simulink model "EMT_ML"  (R2024b)
settings: Solver=ode5  StartTime=0.0  StopTime=200  FixedStep=0.002  RelTol=1e-3
model workspace (MAT data in the model file):
  A = 7.3
  B = 2.71
  C0_shift = 200
  C1_shift = 200
  C2_shift = 200
  Cb = 70
  Cd = 0.6
  EMSInputBus : Simulink.Bus (value not decoded)
  Fb_max = 247500
  JA = 0.4
  JB = 0.4
  JZ = 0.4
  Jc1r2 = 0.01
  Jc3r4 = 0.01
  Jc4 = 0.01
  Je = 2.5
  Jh = 0.01
  Jq1 = 0.01
  Jq2 = 0.01
  Jr1 = 0.01
  Jr3s4 = 0.01
  Js123 = 0.01
  L = 4.472
  NE = [1600 1600 1600 1600 1600 1600 1600 1600 1600 1600 1600 1600 ... (840 elements, 30x28)]
  N_Te = 30
  N_ne = 28
  PE = [0 100.366530527 133.710336161 167.221698607 195.706356687 221.845219395 250.497434286 278.144308305 305.288511886 330.086920096 352.87464656 374.489475338 ... (840 elements, 30x28)]
  PN0 = 0
  Pb_epr = [-45 -45 -40 -30 0 30 40 45 45]
  Pb_max = [0 40 45 45 45]
  Pb_min = [-45 -45 -45 -40 0]
  Pe_ass = 230
  Pe_max = 1103
  Peg = [0 100 120 140 160 180 200 220 240 260 280 300 ... (53 elements, 1x53)]
  R_map = [0.09 0.089 0.09 0.091 0.092 0.093 0.094 0.095 0.096 0.097 0.098]
  SF_C0 = 1.5
  SF_C1 = 1.5
  SF_C2 = 1.5
  SF_Z1 = 1.5
  SF_Z2 = 1.5
  SF_ZD = 1.5
  SOC0 = 60
  SOC_epr = [30 31 50 59 60 61 70 79 80]
  SOC_map = [0 10 20 30 40 50 60 70 80 90 100]
  TA_max_map = [588.855 593.803361345 598.83559322 603.953846154 609.160344828 614.457391304 619.847368421 625.332743363 630.916071429 636.6 642.387272727 648.280733945 ... (115 elements, 1x115)]
  TA_min_map = [-588.855 -593.803361345 -598.83559322 -603.953846154 -609.160344828 -614.457391304 -619.847368421 -625.332743363 -630.916071429 -636.6 -642.387272727 -648.280733945 ... (115 elements, 1x115)]
  TAf = 0
  TB_max_map = [588.855 593.803361345 598.83559322 603.953846154 609.160344828 614.457391304 619.847368421 625.332743363 630.916071429 636.6 642.387272727 648.280733945 ... (115 elements, 1x115)]
  TB_min_map = [-588.855 -593.803361345 -598.83559322 -603.953846154 -609.160344828 -614.457391304 -619.847368421 -625.332743363 -630.916071429 -636.6 -642.387272727 -648.280733945 ... (115 elements, 1x115)]
  TBf = 0
  TE = [0 599 798 998 1168 1324 1495 1660 1822 1970 2106 2235 ... (840 elements, 30x28)]
  TS_A = 0.2
  TS_B = 0.2
  TS_C0 = 0.2
  TS_C1 = 0.2
  TS_C2 = 0.2
  TS_Z = 0.2
  TS_Z1 = 0.2
  TS_Z2 = 0.2
  TS_ZD = 0.2
  TZ_max_map = [537.13125 540.509433962 543.930379747 547.394904459 550.903846154 554.458064516 558.058441558 561.705882353 565.401315789 569.145695364 572.94 576.785234899 ... (131 elements, 1x131)]
  TZ_min_map = [-537.13125 -540.509433962 -543.930379747 -547.394904459 -550.903846154 -554.458064516 -558.058441558 -561.705882353 -565.401315789 -569.145695364 -572.94 -576.785234899 ... (131 elements, 1x131)]
  TZf = 0
  T_generator = [0 185 493.333333333 801.666666667 1110 1418.33333333 1726.66666667]
  T_motor = [0 185 493.333333333 801.666666667 1110 1418.33333333 1726.66666667]
  Te_map = [0 599 798 998 1168 1324 1495 1660 1822 1970 2106 2235 ... (30 elements, 1x30)]
  Te_max = 2754
  Te_max_map = [1168 1324 1495 1660 1822 1970 2106 2235 2355 2458 2543 2606 ... (28 elements, 1x28)]
  Te_start = 1600
  Tef = 100
  Teg = [0 596.8125 636.6 718.741935484 799.916230366 859.41 954.422788606 954.9 996.417391304 1078.98305085 1114.05 1169.26530612 ... (53 elements, 1x53)]
  Temax = 998
  Time = [0 0.1 0.2 0.3 0.4 0.5 0.6 0.7 0.8 0.9 1 1.1 ... (2001 elements, 1x2001)]
  Time_ele = [0 4 8 12 16 20 24 28 32 36 40 44 ... (401 elements, 1x401)]
  Time_fg = [0 2 4 6 8 10 12 14 16 18 20 22 ... (801 elements, 1x801)]
  Tmax_C0 = 2754
  Tmax_C1 = 3505.25455609
  Tmax_C2 = 3505.25455609
  Tmax_Z1 = 5584.80955498
  Tmax_Z2 = 16307.6439005
  Tmax_ZD = 3855.6
  Ts_e = 0.1
  Uoc_map = [814.5 917 933.25 945.75 958.25 969.25 978 985.25 993.25 1003.25 1050]
  V_Shift12 = 32
  V_Shift21 = 25
  V_Start = 10
  Voltage0 = 900
  Voltage_epr = [750 760 900 1000 1050]
  Y_engine = 0.955
  Yc = 0.98
  Yh = 0.96
  Yo = 0.92
  Yq = 0.94
  Z1_shift = 200
  Z2_shift = 200
  a11 = 1.54241568346
  a11_L = 1.54241568346
  a12 = -3.86074191629
  a12_L = 2.43173643789
  a21 = -1.04963112005
  a22 = 2.46948356808
  b11 = 0
  b11_L = 0
  b12 = 3.33
  b12_L = 7.8036
  b21 = 2.23571428571
  b22 = -2.13
  c11 = -0.648333656565
  c12 = 0
  c21 = -0.648333656565
  c22 = 0.680511182109
  controller_id = 1
  controller_name = 'Existing heuristic-grid EMS'
  cycle_grade = [0 0 0 0 0 0 0 0 0 0 0 0 ... (2001 elements, 1x2001)]
  cycle_road = [0.045 0.045 0.045 0.045 0.045 0.045 0.045 0.045 0.045 0.045 0.045 0.045 ... (2001 elements, 1x2001)]
  cycle_steering = [0 0 0 0 0 0 0 0 0 0 0 0 ... (2001 elements, 1x2001)]
  cycle_time = [0 0.1 0.2 0.3 0.4 0.5 0.6 0.7 0.8 0.9 1 1.1 ... (2001 elements, 1x2001)]
  d11 = -0.751666343435
  d12 = 0.3003003003
  d21 = -0.751666343435
  d22 = 0.319488817891
  e11 = -1.54241568346
  e12 = 0
  e21 = 1.04963112005
  e22 = -2.23571428571
  eff_generator = [0.8 0.8 0.79 0.79 0.76 0.74 0.72 0.8 0.85 0.88 0.85 0.8 ... (84 elements, 7x12)]
  eff_motor = [0.8 0.8 0.79 0.79 0.76 0.74 0.72 0.8 0.85 0.88 0.85 0.8 ... (84 elements, 7x12)]
  ele_map = [10 11.46 14.13 19.24 20.94 23.21 20.29 20.23 22.28 17.66 16.24 18.95 ... (401 elements, 1x401)]
  ems_runtime_config : object (value not decoded)
  f11 = -3.86074191629
  f12 = 3.33
  f21 = 2.46948356808
  f22 = -2.13
  fg = 0.045
  fg_map = [0.0125 0.0215 0.0332 0.0452 0.0525 0.0589 0.0584 0.0592 0.0621 0.0576 0.055 0.0572 ... (801 elements, 1x801)]
  fuel_gpkwh = [269.874826377 269.874826377 260.084605263 254.895150301 249.802821062 244.062054381 234.972466555 226.630558735 223.93243551 227.612775381 231.379615385 228.983738255 ... (840 elements, 30x28)]
  fuel_map = [269.874826377 269.874826377 260.084605263 254.895150301 249.802821062 244.062054381 234.972466555 226.630558735 223.93243551 227.612775381 231.379615385 228.983738255 ... (840 elements, 30x28)]
  fuel_map_N = [269.874826377 269.874826377 260.084605263 254.895150301 249.802821062 nan nan nan nan nan nan nan ... (840 elements, 30x28)]
  i = 28
  ic = 4.42
  iq = 1.4
  it = 4
  j = 30
  k1 = 2.13
  k2 = 2.13
  k3 = 2.33
  k4 = 1.92
  kh = 2.88
  kq = 2.17
  kt = 1.83
  mass = 45000
  miu_max = 0.8
  nA_map = [-6000 -5950 -5900 -5850 -5800 -5750 -5700 -5650 -5600 -5550 -5500 -5450 ... (115 elements, 1x115)]
  nA_max = 6000
  nA_min = -6000
  nB_map = [-6000 -5950 -5900 -5850 -5800 -5750 -5700 -5650 -5600 -5550 -5500 -5450 ... (115 elements, 1x115)]
  nB_max = 6000
  nB_min = -6000
  nB_start = 0
  nZ_map = [-8000 -7950 -7900 -7850 -7800 -7750 -7700 -7650 -7600 -7550 -7500 -7450 ... (131 elements, 1x131)]
  nZ_max = 8000
  nZ_min = -8000
  n_generator = [0 318.5 796.25 1274 1751.75 2229.5 2707.25 3185 3662.75 4140.5 4618.25 7007]
  n_motor = [0 318.5 796.25 1274 1751.75 2229.5 2707.25 3185 3662.75 4140.5 4618.25 7007]
  ne_idl = 3000
  ne_map = [1600 1700 1800 1900 2000 2100 2200 2300 2400 2500 2600 2700 ... (28 elements, 1x28)]
  ne_max = 4200
  ne_min = 1600
  ne_start = 200
  neg = [1600 1600 1800 1860 1910 2000 2001 2200 2300 2301 2400 2450 ... (53 elements, 1x53)]
  no_Shift12 = 1589.43589002
  no_Shift21 = 1241.74678908
  rz = 0.318
  startup_feedback_delay_s = 0.002
  startup_power_share = 0.5
  startup_speed_regularizer_rpm = 100
  v_cyc = [0 0 0 0 0 0 0 0 0 0 0 0 ... (2001 elements, 1x2001)]
  voltage_HighA = 1050
  voltage_HighB = 1050
  voltage_HighZ = 1050
  voltage_LowA = 750
  voltage_LowB = 750
  voltage_LowZ = 750
symbols that are objects in the model workspace (value not decoded): ems_runtime_config
undefined symbols (not defined in the file or in its folder): sigbuilder_block
libraries: fl_lib x82, nesl_utility x55, simulink x49, sdl_lib x10, slpidlib x3, simulink_need_slupdate x3, powerlib_extras x1
(part 5 of 7)

== system EMT_ML/Power Coupler /Z2/Z/Z2 ==
  Press : Inport
  Simulink-PS Converter : nesl_utility/Simulink-PS Converter  PhysicalDomain=network_engine_domain  SubClassName=ps_input  LeftPortType=input  RightPortType=output  PseudoPeriodic=off  Frequencies=[]  NoiseDistribution=none  NoiseParameters=[]  Unit=Pa  AffineConversion=off  FilteringAndDerivatives=filter  SimscapeFilterOrder=1  InputFilterTimeConstant=.001  UdotUserProvided=1
  Slip Sensor : Subsystem  mask(Slip Sensor){}
      mask help: The speed unit is r/min.
  Tire Radius2 : Gain  Gain=2500000
  Z2 : sdl_lib/Clutches/Disc Friction Clutch  geometry_model=2  r_eff=130 mm  d_o=189*2 mm  d_i=165.25*2 mm  nS=10  piston_area=0.0264 m^2  unidirectional=0  friction_model=1  mu_w_vector=[ 0 0.1 0.2 0.3 0.4 0.5 1 2 5 10 100 1000 ] rad/s  temperature_TLU=[280.0, 300.0, 320.0] K  mu_static=0.10  mu_static_vector=[0.4, 0.38, 0.36]  mu_coulomb=0.06  mu_coulomb_vector=[ 0.29 0.28 0.26 0.22 0.21 0.2 0.2 0.19 0.19 0.19 0.19 0.19 ]  mu_coulomb_temp_vector=[0.3, 0.28, 0.25]  mu_coulomb_matrix=[0.34, 0.32, 0.3; 0.3, 0.28, 0.25; 0.25, 0.2, 0.15]  mu_interp_method=1  mu_extrap_method=1  d_f=0.6  w_tol=0.001 rad/s  pressure_min=1830 Pa  mu_visc=0.0764 N*m/(rad/s)  initial_state_locked=0  thermal_mass=25 kJ/K  T_init=300 K
      settings: InternalSimscapePortConfiguration="{\"Bottom\":[],\"Left\":[{\"id\":\"P\",\"label\":\"P\",\"type\":\"input\"},{\"id\":\"B\",\"label\":\"B\",\"type\":\"foundation.mechanical.rotational.rotational\"}],\"Right\":[{\"id\":\"F\",\"label\":\"F\",\"type\":\"foundation.mechanical.rotational.rotational\"}],\"Top\":[]}"
  In : PMIOPort  Side=Left
  Out : PMIOPort  Port=2  Side=Right
  r/min : Outport
  wires:
  Slip Sensor/1(r/min) -> r/min/1
  Press/1 -> Tire Radius2/1
  Tire Radius2/1 -> Simulink-PS Converter/1
  connections:
  Slip Sensor/RConn1 -- Out/RConn1 -- Z2/RConn1
  Slip Sensor/LConn1 -- Z2/LConn2 -- In/RConn1
  Simulink-PS Converter/RConn1 -- Z2/LConn1

== system EMT_ML/Vehicle dynamics/vehicle dynamic/vehicle dynamic/Grade Resistance ==
  angle : Inport
  Ground Resistance : Fcn  Expr=0.5*mass*9.8*sin(u)
  Fg : Outport
  wires:
  Ground Resistance/1 -> Fg/1
  angle/1 -> Ground Resistance/1

== system EMT_ML/Vehicle dynamics/vehicle dynamic/vehicle dynamic/Ground Resistance ==
  fg : Inport
  angle : Inport  Port=2
  Ground Resistance : Fcn  Expr=0.5*u(1)*mass*9.8*cos(u(2))
  Mux : Mux  Inputs=2
  Ff : Outport
  wires:
  Ground Resistance/1 -> Ff/1
  Mux/1 -> Ground Resistance/1
  fg/1 -> Mux/1
  angle/1 -> Mux/2

== system EMT_ML/Vehicle dynamics/vehicle dynamic/vehicle dynamic/Mode Judge ==
  v : Inport
  Add : Sum  Inputs=+++
  Compare To Constant1 : simulink/Logic and Bit Operations/Compare To Constant  relop=<  const=-0.1  OutDataTypeStr=uint8
  Compare To Constant2 : simulink/Logic and Bit Operations/Compare To Constant  relop=>  const=0.1  OutDataTypeStr=uint8
  Compare To Constant3 : simulink/Logic and Bit Operations/Compare To Constant  relop=>=  const=-0.1  OutDataTypeStr=uint8
  Compare To Constant4 : simulink/Logic and Bit Operations/Compare To Constant  relop=<=  const=0.1  OutDataTypeStr=uint8
  Data Type Conversion : DataTypeConversion  SaturateOnIntegerOverflow=off  RndMeth=Floor
  Gain : Gain  Gain=3
  Gain1 : Gain  Gain=2
  Gain2 : Gain
  Logical Operator : Logic  AllPortsSameDT=off  OutDataTypeStr=boolean
  F : Outport
  wires:
  Gain1/1 -> Add/2
  Add/1 -> Data Type Conversion/1
  v/1 -> Compare To Constant4/1, Compare To Constant3/1, Compare To Constant2/1, Compare To Constant1/1
  Compare To Constant1/1 -> Gain2/1
  Compare To Constant3/1 -> Logical Operator/1
  Compare To Constant4/1 -> Logical Operator/2
  Compare To Constant2/1 -> Gain1/1
  Logical Operator/1 -> Gain/1
  Data Type Conversion/1 -> F/1
  Gain/1 -> Add/3
  Gain2/1 -> Add/1

== system EMT_ML/Vehicle dynamics/vehicle dynamic/vehicle dynamic/Speed Sensor ==
  Ideal Rotational Motion Sensor : fl_lib/Mechanical/Mechanical Sensors/Ideal Rotational Motion Sensor  reference=foundation.enum.MeasurementReference.difference  acceleration_port=false  velocity_port=true  position_port=true  wrap_angle=false  offset=0 rad
  PS-Simulink Converter : nesl_utility/PS-Simulink Converter  PhysicalDomain=network_engine_domain  SubClassName=ps_output  LeftPortType=input  RightPortType=output  PseudoPeriodic=off  Frequencies=[]  VectorFormat=1-D array  Unit=1  AffineConversion=off
  Reference : fl_lib/Mechanical/Rotational Elements/Mechanical Rotational Reference
  Tire Radius2 : Gain  Gain=30/pi
  shaft : PMIOPort  Side=Left
  r/min : Outport
  wires:
  Tire Radius2/1 -> r/min/1
  PS-Simulink Converter/1 -> Tire Radius2/1
  connections:
  shaft/RConn1 -- Ideal Rotational Motion Sensor/LConn1
  Reference/LConn1 -- Ideal Rotational Motion Sensor/RConn1
  PS-Simulink Converter/LConn1 -- Ideal Rotational Motion Sensor/RConn2

== system EMT_ML/Vehicle dynamics/vehicle dynamic/vehicle dynamic/Steering Resistance ==
  Abs : Abs  SaturateOnIntegerOverflow=off
  Compare To Constant : simulink/Logic and Bit Operations/Compare To Constant  relop=>=  const=10^3  OutDataTypeStr=uint8  ZeroCross=off
  Constant1 : Constant  Value=0
  Memory1 : Memory
  Memory3 : Memory
  Mux : Mux  Inputs=2
  Product2 : Product  RndMeth=Zero
  Sign1 : Signum
  Steering Resistance : Fcn  Expr=miu_max/(0.925+0.15*(u))*mass*9.8*L/4/B
  Switch : Switch  Threshold=1  SaturateOnIntegerOverflow=off  InputSameDT=off
  rou : Fcn  Expr=(u(1)+u(2))/(u(1)-u(2)+0.1^10)/2
  Fs : Outport
  wires:
  Steering Resistance/1 -> Product2/1
  Memory3/1 -> Mux/1
  Memory1/1 -> Mux/2
  Mux/1 -> rou/1
  rou/1 -> Abs/1, Compare To Constant/1, Sign1/1
  Abs/1 -> Steering Resistance/1  "rou"
  Compare To Constant/1 -> Switch/2
  Constant1/1 -> Switch/1
  Switch/1 -> Product2/2
  Sign1/1 -> Switch/3
  Product2/1 -> Fs/1
  [v_Left] -> Memory3/1
  [v_Right] -> Memory1/1

== system EMT_ML/Vehicle dynamics/vehicle dynamic/vehicle dynamic/Torque Actuator ==
  torque : Inport
  Ideal Torque Source : fl_lib/Mechanical/Mechanical Sources/Ideal Torque Source
  Mechanical Rotational Reference : fl_lib/Mechanical/Rotational Elements/Mechanical Rotational Reference
  Simulink-PS Converter : nesl_utility/Simulink-PS Converter  PhysicalDomain=network_engine_domain  SubClassName=ps_input  LeftPortType=input  RightPortType=output  PseudoPeriodic=off  Frequencies=[]  NoiseDistribution=none  NoiseParameters=[]  Unit=1  AffineConversion=off  FilteringAndDerivatives=filter  SimscapeFilterOrder=2  InputFilterTimeConstant=.001  UdotUserProvided=1
  shaft : PMIOPort  Side=Right
  wires:
  torque/1 -> Simulink-PS Converter/1
  connections:
  Simulink-PS Converter/RConn1 -- Ideal Torque Source/RConn1
  Mechanical Rotational Reference/LConn1 -- Ideal Torque Source/RConn2
  shaft/RConn1 -- Ideal Torque Source/LConn1

== system EMT_ML/Vehicle dynamics/vehicle dynamic/vehicle dynamic/Torque Sensor ==
  Ideal Torque Sensor : fl_lib/Mechanical/Mechanical Sensors/Ideal Torque Sensor
  PS-Simulink Converter : nesl_utility/PS-Simulink Converter  PhysicalDomain=network_engine_domain  SubClassName=ps_output  LeftPortType=input  RightPortType=output  PseudoPeriodic=off  Frequencies=[]  VectorFormat=1-D array  Unit=1  AffineConversion=off
  In : PMIOPort  Side=Left
  Out : PMIOPort  Port=2  Side=Right
  Nm : Outport
  wires:
  PS-Simulink Converter/1 -> Nm/1
  connections:
  PS-Simulink Converter/LConn1 -- Ideal Torque Sensor/RConn2
  In/RConn1 -- Ideal Torque Sensor/LConn1
  Ideal Torque Sensor/RConn1 -- Out/RConn1

== system EMT_ML/Vehicle dynamics/vehicle dynamic/vehicle dynamic/Wind Resistance ==
  Air Resistance : Fcn  Expr=0.5*Cd*A*u*u/21.15
  Memory3 : Memory
  Fw : Outport
  wires:
  [v_act] -> Memory3/1
  Memory3/1 -> Air Resistance/1
  Air Resistance/1 -> Fw/1

== system EMT_ML/Vehicle dynamics/vehicle dynamic/vehicle dynamic1/Grade Resistance ==
  angle : Inport
  Ground Resistance : Fcn  Expr=0.5*mass*9.8*sin(u)
  Fg : Outport
  wires:
  angle/1 -> Ground Resistance/1
  Ground Resistance/1 -> Fg/1

== system EMT_ML/Vehicle dynamics/vehicle dynamic/vehicle dynamic1/Ground Resistance ==
  fg : Inport
  angle : Inport  Port=2
  Ground Resistance : Fcn  Expr=0.5*u(1)*mass*9.8*cos(u(2))
  Mux : Mux  Inputs=2
  Ff : Outport
  wires:
  angle/1 -> Mux/2
  fg/1 -> Mux/1
  Mux/1 -> Ground Resistance/1
  Ground Resistance/1 -> Ff/1

== system EMT_ML/Vehicle dynamics/vehicle dynamic/vehicle dynamic1/Mode Judge ==
  v : Inport
  Add : Sum  Inputs=+++
  Compare To Constant1 : simulink/Logic and Bit Operations/Compare To Constant  relop=<  const=-0.1  OutDataTypeStr=uint8
  Compare To Constant2 : simulink/Logic and Bit Operations/Compare To Constant  relop=>  const=0.1  OutDataTypeStr=uint8
  Compare To Constant3 : simulink/Logic and Bit Operations/Compare To Constant  relop=>=  const=-0.1  OutDataTypeStr=uint8
  Compare To Constant4 : simulink/Logic and Bit Operations/Compare To Constant  relop=<=  const=0.1  OutDataTypeStr=uint8
  Data Type Conversion : DataTypeConversion  SaturateOnIntegerOverflow=off  RndMeth=Floor
  Gain : Gain  Gain=3
  Gain1 : Gain  Gain=2
  Gain2 : Gain
  Logical Operator : Logic  AllPortsSameDT=off  OutDataTypeStr=boolean
  F : Outport
  wires:
  Gain2/1 -> Add/1
  Gain/1 -> Add/3
  Data Type Conversion/1 -> F/1
  Logical Operator/1 -> Gain/1
  Compare To Constant2/1 -> Gain1/1
  Compare To Constant4/1 -> Logical Operator/2
  Compare To Constant3/1 -> Logical Operator/1
  Compare To Constant1/1 -> Gain2/1
  v/1 -> Compare To Constant1/1, Compare To Constant2/1, Compare To Constant3/1, Compare To Constant4/1
  Add/1 -> Data Type Conversion/1
  Gain1/1 -> Add/2

== system EMT_ML/Vehicle dynamics/vehicle dynamic/vehicle dynamic1/Speed Sensor ==
  Ideal Rotational Motion Sensor : fl_lib/Mechanical/Mechanical Sensors/Ideal Rotational Motion Sensor  reference=foundation.enum.MeasurementReference.difference  acceleration_port=false  velocity_port=true  position_port=true  wrap_angle=false  offset=0 rad
  PS-Simulink Converter : nesl_utility/PS-Simulink Converter  PhysicalDomain=network_engine_domain  SubClassName=ps_output  LeftPortType=input  RightPortType=output  PseudoPeriodic=off  Frequencies=[]  VectorFormat=1-D array  Unit=1  AffineConversion=off
  Reference : fl_lib/Mechanical/Rotational Elements/Mechanical Rotational Reference
  Tire Radius2 : Gain  Gain=30/pi
  shaft : PMIOPort  Side=Left
  r/min : Outport
  wires:
  PS-Simulink Converter/1 -> Tire Radius2/1
  Tire Radius2/1 -> r/min/1
  connections:
  PS-Simulink Converter/LConn1 -- Ideal Rotational Motion Sensor/RConn2
  Reference/LConn1 -- Ideal Rotational Motion Sensor/RConn1
  shaft/RConn1 -- Ideal Rotational Motion Sensor/LConn1

== system EMT_ML/Vehicle dynamics/vehicle dynamic/vehicle dynamic1/Steering Resistance ==
  Abs : Abs  SaturateOnIntegerOverflow=off
  Compare To Constant : simulink/Logic and Bit Operations/Compare To Constant  relop=>=  const=10^3  OutDataTypeStr=uint8  ZeroCross=off
  Constant1 : Constant  Value=0
  Memory1 : Memory
  Memory3 : Memory
  Mux : Mux  Inputs=2
  Product2 : Product  RndMeth=Zero
  Sign1 : Signum
  Steering Resistance : Fcn  Expr=miu_max/(0.925+0.15*(u))*mass*9.8*L/4/B
  Switch : Switch  Threshold=1  SaturateOnIntegerOverflow=off  InputSameDT=off
  rou : Fcn  Expr=(u(1)+u(2))/(u(2)-u(1)+0.1^10)/2
  Fs : Outport
  wires:
  [v_Right] -> Memory1/1
  [v_Left] -> Memory3/1
  Product2/1 -> Fs/1
  Sign1/1 -> Switch/3
  Switch/1 -> Product2/2
  Constant1/1 -> Switch/1
  Compare To Constant/1 -> Switch/2
  Abs/1 -> Steering Resistance/1  "rou"
  rou/1 -> Sign1/1, Compare To Constant/1, Abs/1
  Mux/1 -> rou/1
  Memory1/1 -> Mux/2
  Memory3/1 -> Mux/1
  Steering Resistance/1 -> Product2/1

== system EMT_ML/Vehicle dynamics/vehicle dynamic/vehicle dynamic1/Torque Actuator ==
  torque : Inport
  Ideal Torque Source : fl_lib/Mechanical/Mechanical Sources/Ideal Torque Source
  Mechanical Rotational Reference : fl_lib/Mechanical/Rotational Elements/Mechanical Rotational Reference
  Simulink-PS Converter : nesl_utility/Simulink-PS Converter  PhysicalDomain=network_engine_domain  SubClassName=ps_input  LeftPortType=input  RightPortType=output  PseudoPeriodic=off  Frequencies=[]  NoiseDistribution=none  NoiseParameters=[]  Unit=1  AffineConversion=off  FilteringAndDerivatives=filter  SimscapeFilterOrder=2  InputFilterTimeConstant=.001  UdotUserProvided=1
  shaft : PMIOPort  Side=Right
  wires:
  torque/1 -> Simulink-PS Converter/1
  connections:
  shaft/RConn1 -- Ideal Torque Source/LConn1
  Mechanical Rotational Reference/LConn1 -- Ideal Torque Source/RConn2
  Simulink-PS Converter/RConn1 -- Ideal Torque Source/RConn1

== system EMT_ML/Vehicle dynamics/vehicle dynamic/vehicle dynamic1/Torque Sensor ==
  Ideal Torque Sensor : fl_lib/Mechanical/Mechanical Sensors/Ideal Torque Sensor
  PS-Simulink Converter : nesl_utility/PS-Simulink Converter  PhysicalDomain=network_engine_domain  SubClassName=ps_output  LeftPortType=input  RightPortType=output  PseudoPeriodic=off  Frequencies=[]  VectorFormat=1-D array  Unit=1  AffineConversion=off
  In : PMIOPort  Side=Left
  Out : PMIOPort  Port=2  Side=Right
  Nm : Outport
  wires:
  PS-Simulink Converter/1 -> Nm/1
  connections:
  Ideal Torque Sensor/RConn1 -- Out/RConn1
  In/RConn1 -- Ideal Torque Sensor/LConn1
  PS-Simulink Converter/LConn1 -- Ideal Torque Sensor/RConn2

== system EMT_ML/Vehicle dynamics/vehicle dynamic/vehicle dynamic1/Wind Resistance ==
  Air Resistance : Fcn  Expr=0.5*Cd*A*u*u/21.15
  Memory3 : Memory
  Fw : Outport
  wires:
  [v_act] -> Memory3/1
  Memory3/1 -> Air Resistance/1
  Air Resistance/1 -> Fw/1

== system EMT_ML/engine/Engine/Subsystem1/Torque Actuator ==
  torque : Inport
  Ideal Torque Source : fl_lib/Mechanical/Mechanical Sources/Ideal Torque Source
  Mechanical Rotational Reference : fl_lib/Mechanical/Rotational Elements/Mechanical Rotational Reference
  Simulink-PS Converter : nesl_utility/Simulink-PS Converter  PhysicalDomain=network_engine_domain  SubClassName=ps_input  LeftPortType=input  RightPortType=output  PseudoPeriodic=off  Frequencies=[]  NoiseDistribution=none  NoiseParameters=[]  Unit=N*m  AffineConversion=off  FilteringAndDerivatives=zero  SimscapeFilterOrder=1  InputFilterTimeConstant=.001  UdotUserProvided=0
  shaft : PMIOPort  Side=Right
  wires:
  torque/1 -> Simulink-PS Converter/1
  connections:
  Simulink-PS Converter/RConn1 -- Ideal Torque Source/RConn1
  Mechanical Rotational Reference/LConn1 -- Ideal Torque Source/RConn2
  shaft/RConn1 -- Ideal Torque Source/LConn1

== system EMT_ML/motorA/Motor/Mechanical Body/Max & Min Torque Control ==
  speed : Inport
  Tm_com : Inport  Port=2
  Lookup Table : Lookup  InputValues=nm_map  Table=Tm_max_map  SaturateOnIntegerOverflow=off
  Lookup Table1 : Lookup  InputValues=nm_map  Table=Tm_min_map  SaturateOnIntegerOverflow=off
  Saturation Dynamic : simulink/Discontinuities/Saturation Dynamic  OutMin=[]  OutMax=[]  OutDataTypeStr=Inherit: Same as second input  OutDataType=sfix(16)  OutScaling=2^-10  DoSatur=off
  Saturation1 : Saturate  UpperLimit=max(nm_map)  LowerLimit=min(nm_map)
  Saturation2 : Saturate  UpperLimit=max(nm_map)  LowerLimit=min(nm_map)
  Transfer Fcn : TransferFcn  Denominator=[T 1]
  torque : Outport
  wires:
  speed/1 -> Saturation2/1, Saturation1/1
  Lookup Table/1 -> Saturation Dynamic/1
  Lookup Table1/1 -> Saturation Dynamic/3
  Saturation1/1 -> Lookup Table/1
  Saturation2/1 -> Lookup Table1/1
  Tm_com/1 -> Saturation Dynamic/2
  Saturation Dynamic/1 -> Transfer Fcn/1
  Transfer Fcn/1 -> torque/1

== system EMT_ML/motorA/Motor/Mechanical Body/Resistance ==
  speed : Inport
  Constant2 : Constant  Value=-Tmf
  Product2 : Product  RndMeth=Zero
  Sign2 : Signum
  Torque Actuator : Subsystem  mask(Torque Actuator){}
      mask help: The torque unit is Nm.
  Tmf : PMIOPort  Side=Right
  wires:
  speed/1 -> Sign2/1
  Product2/1 -> Torque Actuator/1(torque)
  Sign2/1 -> Product2/1
  Constant2/1 -> Product2/2
  connections:
  Tmf/RConn1 -- Torque Actuator/RConn1

== system EMT_ML/motorA/Motor/Mechanical Body/Speed Sensor ==
  Ideal Rotational Motion Sensor : fl_lib/Mechanical/Mechanical Sensors/Ideal Rotational Motion Sensor  reference=foundation.enum.MeasurementReference.difference  acceleration_port=false  velocity_port=true  position_port=true  wrap_angle=false  offset=0 rad
  PS-Simulink Converter : nesl_utility/PS-Simulink Converter  PhysicalDomain=network_engine_domain  SubClassName=ps_output  LeftPortType=input  RightPortType=output  PseudoPeriodic=off  Frequencies=[]  VectorFormat=1-D array  Unit=rad/s  AffineConversion=off
  Reference : fl_lib/Mechanical/Rotational Elements/Mechanical Rotational Reference
  Tire Radius2 : Gain  Gain=30/pi
  shaft : PMIOPort  Side=Left
  r/min : Outport
  wires:
  Tire Radius2/1 -> r/min/1
  PS-Simulink Converter/1 -> Tire Radius2/1
  connections:
  shaft/RConn1 -- Ideal Rotational Motion Sensor/LConn1
  Reference/LConn1 -- Ideal Rotational Motion Sensor/RConn1
  PS-Simulink Converter/LConn1 -- Ideal Rotational Motion Sensor/RConn2

== system EMT_ML/motorA/Motor/Mechanical Body/Torque Actuator ==
  torque : Inport
  Ideal Torque Source : fl_lib/Mechanical/Mechanical Sources/Ideal Torque Source
  Mechanical Rotational Reference : fl_lib/Mechanical/Rotational Elements/Mechanical Rotational Reference
  Simulink-PS Converter : nesl_utility/Simulink-PS Converter  PhysicalDomain=network_engine_domain  SubClassName=ps_input  LeftPortType=input  RightPortType=output  PseudoPeriodic=off  Frequencies=[]  NoiseDistribution=none  NoiseParameters=[]  Unit=N*m  AffineConversion=off  FilteringAndDerivatives=filter  SimscapeFilterOrder=1  InputFilterTimeConstant=.001  UdotUserProvided=1
  shaft : PMIOPort  Side=Right
  wires:
  torque/1 -> Simulink-PS Converter/1
  connections:
  shaft/RConn1 -- Ideal Torque Source/LConn1
  Mechanical Rotational Reference/LConn1 -- Ideal Torque Source/RConn2
  Simulink-PS Converter/RConn1 -- Ideal Torque Source/RConn1

== system EMT_ML/motorB/Motor/Mechanical Body/Max & Min Speed Control ==
  speed : Inport
  Tm_com : Inport  Port=2
  Lookup Table : Lookup  InputValues=nm_map  Table=Tm_max_map  SaturateOnIntegerOverflow=off
  Lookup Table1 : Lookup  InputValues=nm_map  Table=Tm_min_map  SaturateOnIntegerOverflow=off
  Saturation Dynamic : simulink/Discontinuities/Saturation Dynamic  OutMin=[]  OutMax=[]  OutDataTypeStr=Inherit: Same as second input  OutDataType=sfix(16)  OutScaling=2^-10  DoSatur=off
  Saturation1 : Saturate  UpperLimit=max(nm_map)  LowerLimit=min(nm_map)
  Saturation2 : Saturate  UpperLimit=max(nm_map)  LowerLimit=min(nm_map)
  Transfer Fcn : TransferFcn  Denominator=[T 1]
  torque : Outport
  wires:
  Transfer Fcn/1 -> torque/1
  speed/1 -> Saturation2/1, Saturation1/1
  Lookup Table/1 -> Saturation Dynamic/1
  Lookup Table1/1 -> Saturation Dynamic/3
  Saturation1/1 -> Lookup Table/1
  Saturation2/1 -> Lookup Table1/1
  Tm_com/1 -> Saturation Dynamic/2
  Saturation Dynamic/1 -> Transfer Fcn/1

== system EMT_ML/motorB/Motor/Mechanical Body/Resistance ==
  speed : Inport
  Constant2 : Constant  Value=-Tmf
  Product2 : Product  RndMeth=Zero
  Sign2 : Signum
  Torque Actuator : Subsystem  mask(Torque Actuator){}
      mask help: The torque unit is Nm.
  Tmf : PMIOPort  Side=Right
  wires:
  speed/1 -> Sign2/1
  Product2/1 -> Torque Actuator/1(torque)
  Sign2/1 -> Product2/1
  Constant2/1 -> Product2/2
  connections:
  Tmf/RConn1 -- Torque Actuator/RConn1

== system EMT_ML/motorB/Motor/Mechanical Body/Speed Sensor ==
  Ideal Rotational Motion Sensor : fl_lib/Mechanical/Mechanical Sensors/Ideal Rotational Motion Sensor  reference=foundation.enum.MeasurementReference.difference  acceleration_port=false  velocity_port=true  position_port=true  wrap_angle=false  offset=0 rad
  PS-Simulink Converter : nesl_utility/PS-Simulink Converter  PhysicalDomain=network_engine_domain  SubClassName=ps_output  LeftPortType=input  RightPortType=output  PseudoPeriodic=off  Frequencies=[]  VectorFormat=1-D array  Unit=rad/s  AffineConversion=off
  Reference : fl_lib/Mechanical/Rotational Elements/Mechanical Rotational Reference
  Tire Radius2 : Gain  Gain=30/pi
  shaft : PMIOPort  Side=Left
  r/min : Outport
  wires:
  Tire Radius2/1 -> r/min/1
  PS-Simulink Converter/1 -> Tire Radius2/1
  connections:
  shaft/RConn1 -- Ideal Rotational Motion Sensor/LConn1
  Reference/LConn1 -- Ideal Rotational Motion Sensor/RConn1
  PS-Simulink Converter/LConn1 -- Ideal Rotational Motion Sensor/RConn2

== system EMT_ML/motorB/Motor/Mechanical Body/Torque Actuator ==
  torque : Inport
  Ideal Torque Source : fl_lib/Mechanical/Mechanical Sources/Ideal Torque Source
  Mechanical Rotational Reference : fl_lib/Mechanical/Rotational Elements/Mechanical Rotational Reference
  Simulink-PS Converter : nesl_utility/Simulink-PS Converter  PhysicalDomain=network_engine_domain  SubClassName=ps_input  LeftPortType=input  RightPortType=output  PseudoPeriodic=off  Frequencies=[]  NoiseDistribution=none  NoiseParameters=[]  Unit=N*m  AffineConversion=off  FilteringAndDerivatives=filter  SimscapeFilterOrder=1  InputFilterTimeConstant=.001  UdotUserProvided=1
  shaft : PMIOPort  Side=Right
  wires:
  torque/1 -> Simulink-PS Converter/1
  connections:
  shaft/RConn1 -- Ideal Torque Source/LConn1
  Mechanical Rotational Reference/LConn1 -- Ideal Torque Source/RConn2
  Simulink-PS Converter/RConn1 -- Ideal Torque Source/RConn1

== system EMT_ML/Control Unit/Control/EVT1_H Stage/clutches condition/Subsystem ==
  Constant1 : Constant
  C0 : Outport
  wires:
  Constant1/1 -> C0/1

== system EMT_ML/Control Unit/Control/EVT1_H Stage/clutches condition/Subsystem1 ==
  Constant1 : Constant
  Z2 : Outport
  wires:
  Constant1/1 -> Z2/1

== system EMT_ML/Control Unit/Control/EVT1_H Stage/clutches condition/Subsystem2 ==
  Compare To Constant1 : simulink/Logic and Bit Operations/Compare To Constant  relop=<  const=C1_shift  OutDataTypeStr=uint8
  Data Type Conversion : DataTypeConversion  SaturateOnIntegerOverflow=off  RndMeth=Floor
  Fcn : Fcn  Expr=V_Shift12+5*(u-1)
  Logical Operator1 : Logic  AllPortsSameDT=off  OutDataTypeStr=boolean
  Memory1 : Memory
  Memory2 : Memory
  Memory5 : Memory
  Relational Operator : RelationalOperator  OutDataTypeStr=boolean  InputSameDT=off
  C1 : Outport
  wires:
  Logical Operator1/1 -> Data Type Conversion/1
  Compare To Constant1/1 -> Logical Operator1/2
  Relational Operator/1 -> Logical Operator1/1
  Fcn/1 -> Relational Operator/2
  Memory1/1 -> Fcn/1
  [Acc_pedal] -> Memory1/1
  Memory2/1 -> Relational Operator/1
  Memory5/1 -> Compare To Constant1/1
  [C1_rela] -> Memory5/1
  Data Type Conversion/1 -> C1/1
  [v_act] -> Memory2/1

== system EMT_ML/Control Unit/Control/EVT1_H Stage/clutches condition/Subsystem4 ==
  Constant1 : Constant  Value=0
  Z1 : Outport
  wires:
  Constant1/1 -> Z1/1

== system EMT_ML/Control Unit/Control/EVT1_H Stage/engine torque/Subsystem1 ==
  Te_ref : Inport
  ne_act : Inport  Port=2
  Constant : Constant  Value=ne_idl
  Constant1 : Constant  Value=0
  Lookup Table : Lookup  InputValues=ne_map  Table=Te_max_map  SaturateOnIntegerOverflow=off
  Memory1 : Memory
  Memory5 : Memory
  PID Controller2 : slpidlib/PID Controller  Controller=PID  Form=Parallel  TimeDomain=Continuous-time  UseExternalTs=off  SampleTime=-1  IntegratorMethod=Forward Euler  FilterMethod=Forward Euler  ControllerParametersSource=internal  P=4  I=0.01  UseKiTs=off  D=10  UseExternalDerivativeSource=off  N=100  UseFilter=on  TunerSelectOption=Transfer Function Based (PID Tuner App)  InitialConditionSource=internal  InitialConditionForIntegrator=0  InitialConditionForFilter=0  DifferentiatorICPrevScaledInput=0  ExternalReset=none  TrackingMode=off  Kt=1  LimitOutput=off  SatLimitsSource=internal  UpperSaturationLimit=inf  LowerSaturationLimit=-inf  LinearizeAsGain=on  AntiWindupMode=none  Kb=1  LimitIntegrator=off  UpperIntegratorSaturationLimit=inf  LowerIntegratorSaturationLimit=-inf  POutMin=[]  POutMax=[]  IOutMin=[]  IOutMax=[]  DOutMin=[]  DOutMax=[]  NOutMin=[]  NOutMax=[]  SumOutMin=[]  SumOutMax=[]  SaturationOutMin=[]  SaturationOutMax=[]  PParamMin=[]  PParamMax=[]  IParamMin=[]  IParamMax=[]  DParamMin=[]  DParamMax=[]  NParamMin=[]  NParamMax=[]  KbParamMin=[]  KbParamMax=[]  KtParamMin=[]  KtParamMax=[]  KbOutMin=[]  KbOutMax=[]  KtOutMin=[]  KtOutMax=[]  IntegratorOutMin=[]  IntegratorOutMax=[]  FilterOutMin=[]  FilterOutMax=[]  SumI1OutMin=[]  SumI1OutMax=[]  SumI2OutMin=[]  SumI2OutMax=[]  SumI3OutMin=[]  SumI3OutMax=[]  SumI4OutMin=[]  SumI4OutMax=[]  SumDOutMin=[]  SumDOutMax=[]  DifferentiatorOutMin=[]  DifferentiatorOutMax=[]  FilterDiffOutCoefMin=[]  FilterDiffOutCoefMax=[]  ReciprocalOutMin=[]  ReciprocalOutMax=[]  SumDenOutMin=[]  SumDenOutMax=[]  SumNumOutMin=[]  SumNumOutMax=[]  DivideOutMin=[]  DivideOutMax=[]  UdiffTsProdOutMin=[]  UdiffTsProdOutMax=[]  NTsProdOutMin=[]  NTsProdOutMax=[]  UintegralTsProdOutMin=[]  UintegralTsProdOutMax=[]  UngainTsProdOutMin=[]  UngainTsProdOutMax=[]  ClampingZeroOutDataTypeStr=Inherit: Inherit via back propagation  ClampingZeroOutMin=[]  ClampingZeroOutMax=[]  FilterDenConstantOutDataTypeStr=Inherit: Inherit via back propagation  FilterDenConstantOutMin=[]  FilterDenConstantOutMax=[]  PCopyOutDataTypeStr=Inherit: Inherit via back propagation  PCopyOutMin=[]  PCopyOutMax=[]  NCopyOutDataTypeStr=Inherit: Inherit via back propagation  NCopyOutMin=[]  NCopyOutMax=[]  IntegratorContinuousStateAttributes=''  IntegratorStateMustResolveToSignalObject=off  IntegratorRTWStateStorageClass=Auto  FilterContinuousStateAttributes=''  FilterStateMustResolveToSignalObject=off  FilterRTWStateStorageClass=Auto  ParallelPVariant=InternalParameters  IdealPVariant=Disabled  IVariant=InternalParameters  DVariant=InternalParameters  IntegratorVariant=Continuous  SatVariant=Disabled  AWVariant=Passthrough  PCopyVariant=Disabled  TRVariant=Disabled  FdbkBlocksVariant=Forward  IdealPFdbkVariant=Disabled  SatFdbkVariant=Disabled  DerivativeFilterVariant=ContFilter  NVariant=InternalParameters  NCopyVariant=Disabled  FilterICVariant=InternalICsFilter  IntegratorICVariant=InternalICs  ExternalResetVariant=Disabled  TRSumVariant=Passthrough  SumFdbkVariant=Disabled  SumVariant=Sum_PID  TsampFilterVariant=InternalTs  TsampNgainVariant=Passthrough  TsampIntegralVariant=Disabled_SignalSpec  ExternalSaturationOutDataTypeStr=Inherit: Same as second input  DerivativeSourceVariant=ErrorSignal  PreIntVariant=InternalPreInt
  Saturation : Saturate  UpperLimit=max(ne_map)  LowerLimit=min(ne_map)
  Saturation Dynamic : simulink/Discontinuities/Saturation Dynamic  OutMin=[]  OutMax=[]  OutDataTypeStr=Inherit: Same as second input  OutDataType=sfix(16)  OutScaling=2^-10  DoSatur=off
  Sum1 : Sum  Inputs=+-
  Switch : Switch  Criteria=u2 > Threshold  Threshold=10  SaturateOnIntegerOverflow=off  InputSameDT=off
  ne_act1 : InportShadow  Port=2
  Te_com : Outport
  wires:
  Memory1/1 -> Saturation/1
  ne_act1/1 -> Memory1/1
  Switch/1 -> Saturation Dynamic/2
  Saturation Dynamic/1 -> Te_com/1
  Constant1/1 -> Saturation Dynamic/3
  Lookup Table/1 -> Saturation Dynamic/1
  Saturation/1 -> Lookup Table/1
  Constant/1 -> Sum1/1
  Te_ref/1 -> Switch/2, Switch/1
  ne_act/1 -> Memory5/1
  Memory5/1 -> Sum1/2
  Sum1/1 -> PID Controller2/1
  PID Controller2/1 -> Switch/3

== system EMT_ML/Control Unit/Control/EVT2 Stage/clutches condition/Subsystem ==
  Constant1 : Constant
  C0 : Outport
  wires:
  Constant1/1 -> C0/1

== system EMT_ML/Control Unit/Control/EVT2 Stage/clutches condition/Subsystem1 ==
  Compare To Constant1 : simulink/Logic and Bit Operations/Compare To Constant  relop=<  const=Z2_shift  OutDataTypeStr=uint8
  Data Type Conversion1 : DataTypeConversion  SaturateOnIntegerOverflow=off  RndMeth=Floor
  Fcn : Fcn  Expr=V_Shift21+5*u
  Logical Operator1 : Logic  AllPortsSameDT=off  OutDataTypeStr=boolean
  Memory1 : Memory
  Memory2 : Memory
  Memory5 : Memory
  Relational Operator : RelationalOperator  Operator=<=  OutDataTypeStr=boolean  InputSameDT=off
  Z2 : Outport
  wires:
  Fcn/1 -> Relational Operator/2
  Memory1/1 -> Fcn/1
  [Acc_pedal] -> Memory1/1
  Data Type Conversion1/1 -> Z2/1
  Logical Operator1/1 -> Data Type Conversion1/1
  Compare To Constant1/1 -> Logical Operator1/2
  Relational Operator/1 -> Logical Operator1/1
  [v_act] -> Memory2/1
  Memory2/1 -> Relational Operator/1
  [Z2_rela] -> Memory5/1
  Memory5/1 -> Compare To Constant1/1

== system EMT_ML/Control Unit/Control/EVT2 Stage/clutches condition/Subsystem2 ==
  Constant1 : Constant
  C1 : Outport
  wires:
  Constant1/1 -> C1/1

== system EMT_ML/Control Unit/Control/EVT2 Stage/clutches condition/Subsystem4 ==
  Constant1 : Constant  Value=0
  Z1 : Outport
  wires:
  Constant1/1 -> Z1/1

== system EMT_ML/Control Unit/Control/EVT2 Stage/motorZ torque/Subsystem1 ==
  nZ_act : Inport
  Constant3 : Constant  Value=0
  Memory5 : Memory
  PID Controller2 : slpidlib/PID Controller  Controller=PID  Form=Parallel  TimeDomain=Continuous-time  UseExternalTs=off  SampleTime=-1  IntegratorMethod=Forward Euler  FilterMethod=Forward Euler  ControllerParametersSource=internal  P=2  I=0.01  UseKiTs=off  D=0.1  UseExternalDerivativeSource=off  N=100  UseFilter=on  TunerSelectOption=Transfer Function Based (PID Tuner App)  InitialConditionSource=internal  InitialConditionForIntegrator=0  InitialConditionForFilter=0  DifferentiatorICPrevScaledInput=0  ExternalReset=none  TrackingMode=off  Kt=1  LimitOutput=off  SatLimitsSource=internal  UpperSaturationLimit=inf  LowerSaturationLimit=-inf  LinearizeAsGain=on  AntiWindupMode=none  Kb=1  LimitIntegrator=off  UpperIntegratorSaturationLimit=inf  LowerIntegratorSaturationLimit=-inf  POutMin=[]  POutMax=[]  IOutMin=[]  IOutMax=[]  DOutMin=[]  DOutMax=[]  NOutMin=[]  NOutMax=[]  SumOutMin=[]  SumOutMax=[]  SaturationOutMin=[]  SaturationOutMax=[]  PParamMin=[]  PParamMax=[]  IParamMin=[]  IParamMax=[]  DParamMin=[]  DParamMax=[]  NParamMin=[]  NParamMax=[]  KbParamMin=[]  KbParamMax=[]  KtParamMin=[]  KtParamMax=[]  KbOutMin=[]  KbOutMax=[]  KtOutMin=[]  KtOutMax=[]  IntegratorOutMin=[]  IntegratorOutMax=[]  FilterOutMin=[]  FilterOutMax=[]  SumI1OutMin=[]  SumI1OutMax=[]  SumI2OutMin=[]  SumI2OutMax=[]  SumI3OutMin=[]  SumI3OutMax=[]  SumI4OutMin=[]  SumI4OutMax=[]  SumDOutMin=[]  SumDOutMax=[]  DifferentiatorOutMin=[]  DifferentiatorOutMax=[]  FilterDiffOutCoefMin=[]  FilterDiffOutCoefMax=[]  ReciprocalOutMin=[]  ReciprocalOutMax=[]  SumDenOutMin=[]  SumDenOutMax=[]  SumNumOutMin=[]  SumNumOutMax=[]  DivideOutMin=[]  DivideOutMax=[]  UdiffTsProdOutMin=[]  UdiffTsProdOutMax=[]  NTsProdOutMin=[]  NTsProdOutMax=[]  UintegralTsProdOutMin=[]  UintegralTsProdOutMax=[]  UngainTsProdOutMin=[]  UngainTsProdOutMax=[]  ClampingZeroOutDataTypeStr=Inherit: Inherit via back propagation  ClampingZeroOutMin=[]  ClampingZeroOutMax=[]  FilterDenConstantOutDataTypeStr=Inherit: Inherit via back propagation  FilterDenConstantOutMin=[]  FilterDenConstantOutMax=[]  PCopyOutDataTypeStr=Inherit: Inherit via back propagation  PCopyOutMin=[]  PCopyOutMax=[]  NCopyOutDataTypeStr=Inherit: Inherit via back propagation  NCopyOutMin=[]  NCopyOutMax=[]  IntegratorContinuousStateAttributes=''  IntegratorStateMustResolveToSignalObject=off  IntegratorRTWStateStorageClass=Auto  FilterContinuousStateAttributes=''  FilterStateMustResolveToSignalObject=off  FilterRTWStateStorageClass=Auto  ParallelPVariant=InternalParameters  IdealPVariant=Disabled  IVariant=InternalParameters  DVariant=InternalParameters  IntegratorVariant=Continuous  SatVariant=Disabled  AWVariant=Passthrough  PCopyVariant=Disabled  TRVariant=Disabled  FdbkBlocksVariant=Forward  IdealPFdbkVariant=Disabled  SatFdbkVariant=Disabled  DerivativeFilterVariant=ContFilter  NVariant=InternalParameters  NCopyVariant=Disabled  FilterICVariant=InternalICsFilter  IntegratorICVariant=InternalICs  ExternalResetVariant=Disabled  TRSumVariant=Passthrough  SumFdbkVariant=Disabled  SumVariant=Sum_PID  TsampFilterVariant=InternalTs  TsampNgainVariant=Passthrough  TsampIntegralVariant=Disabled_SignalSpec  ExternalSaturationOutDataTypeStr=Inherit: Same as second input  DerivativeSourceVariant=ErrorSignal  PreIntVariant=InternalPreInt
  Sum1 : Sum  Inputs=+-
  TZ_com : Outport
  wires:
  Memory5/1 -> Sum1/2
  Constant3/1 -> Sum1/1
  nZ_act/1 -> Memory5/1
  Sum1/1 -> PID Controller2/1
  PID Controller2/1 -> TZ_com/1

== system EMT_ML/Control Unit/Control/Power Distribution/Electric Power Requirement/Data ==
  PN_com : Inport
  PN_max : Inport  Port=2
  PN_min : Inport  Port=3
  tag scope: PN_com=global, PN_max=global, PN_min=global
  wires:
  PN_min/1 -> [PN_min]
  PN_max/1 -> [PN_max]
  PN_com/1 -> [PN_com]

== system EMT_ML/Control Unit/Control/Power Distribution/Feasible Control Range/State Calculation ==
  s : Inport
  ne : Inport  Port=2
  v_act : Inport  Port=3
  Speed : Subsystem
  Subsystem3 : Subsystem
  no1 : Fcn  Expr=u*(1+kh)/kh*ic/0.377/rz
  stage : Outport
  ne_act : Outport  Port=2
  nA_act : Outport  Port=3
  nB_act : Outport  Port=4
  no_act : Outport  Port=5
  wires:
  Speed/2(nB) -> nB_act/1
  Speed/1(nA) -> nA_act/1
  ne/1 -> ne_act/1, Speed/2(ne)
  no1/1 -> no_act/1, Speed/3(no)
  Subsystem3/1(1) -> Speed/1(stage)
  s/1 -> stage/1, Subsystem3/1(0)
  v_act/1 -> no1/1

== system EMT_ML/Control Unit/Control/Power Distribution/Feasible Control Range/State Predition ==
  stage : Inport
  ne_act : Inport  Port=2
  nA_act : Inport  Port=3
  nB_act : Inport  Port=4
  no_act : Inport  Port=5
  TA Range : Subsystem
  TB Range : Subsystem
  Te Range : Subsystem
  Z : Subsystem
  ne_act2 : InportShadow  Port=2
  stage_k : Outport
  ne_k : Outport  Port=2
  no_k : Outport  Port=3
  Te_k : Outport  Port=4
  TA_k : Outport  Port=5
  TB_k : Outport  Port=6
  wires:
  ne_act/1 -> Te Range/1(ne_act)
  Te Range/1(Te_k) -> Te_k/1
  nA_act/1 -> TA Range/1(nA)
  TA Range/1(TA_R) -> TA_k/1
  nB_act/1 -> TB Range/1(nB)
  TB Range/1(TB_R) -> TB_k/1
  Z/1(ne_k) -> ne_k/1
  stage/1 -> Z/1(stage), stage_k/1
  ne_act2/1 -> Z/2(ne_act)
  no_act/1 -> Z/3(no_act), no_k/1

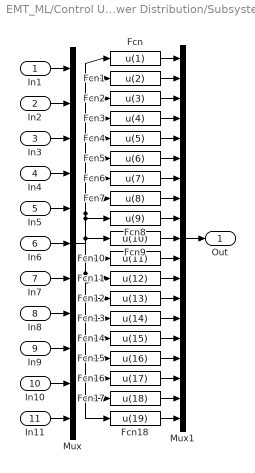
== system EMT_ML/Control Unit/Control/Power Distribution/Optimal Power Distribution/Subsystem ==
  In1 : Inport
  In2 : Inport  Port=2
  In3 : Inport  Port=3
  In4 : Inport  Port=4
  In5 : Inport  Port=5
  In6 : Inport  Port=6
  In7 : Inport  Port=7
  In8 : Inport  Port=8
  In9 : Inport  Port=9
  In10 : Inport  Port=10
  In11 : Inport  Port=11
  Fcn : Fcn  Expr=u(1)
  Fcn1 : Fcn  Expr=u(2)
  Fcn10 : Fcn  Expr=u(11)
  Fcn11 : Fcn  Expr=u(12)
  Fcn12 : Fcn  Expr=u(13)
  Fcn13 : Fcn  Expr=u(14)
  Fcn14 : Fcn  Expr=u(15)
  Fcn15 : Fcn  Expr=u(16)
  Fcn16 : Fcn  Expr=u(17)
  Fcn17 : Fcn  Expr=u(18)
  Fcn18 : Fcn  Expr=u(19)
  Fcn2 : Fcn  Expr=u(3)
  Fcn3 : Fcn  Expr=u(4)
  Fcn4 : Fcn  Expr=u(5)
  Fcn5 : Fcn  Expr=u(6)
  Fcn6 : Fcn  Expr=u(7)
  Fcn7 : Fcn  Expr=u(8)
  Fcn8 : Fcn  Expr=u(9)
  Fcn9 : Fcn  Expr=u(10)
  Mux : Mux  Inputs=11
  Mux1 : Mux  Inputs=19
  Out : Outport
  wires:
  In9/1 -> Mux/9
  In8/1 -> Mux/8
  In7/1 -> Mux/7
  Mux1/1 -> Out/1
  In6/1 -> Mux/6
  In5/1 -> Mux/5
  In4/1 -> Mux/4
  In3/1 -> Mux/3
  In2/1 -> Mux/2
  In1/1 -> Mux/1
  Fcn15/1 -> Mux1/16
  Fcn14/1 -> Mux1/15
  Fcn13/1 -> Mux1/14
  Fcn12/1 -> Mux1/13
  Fcn11/1 -> Mux1/12
  Fcn10/1 -> Mux1/11
  Fcn9/1 -> Mux1/10
  Fcn8/1 -> Mux1/9
  Fcn7/1 -> Mux1/8
  Fcn6/1 -> Mux1/7
  Fcn5/1 -> Mux1/6
  Fcn4/1 -> Mux1/5
  Fcn3/1 -> Mux1/4
  Fcn2/1 -> Mux1/3
  Fcn1/1 -> Mux1/2
  Fcn/1 -> Mux1/1
  In10/1 -> Mux/10
  Fcn16/1 -> Mux1/17
  Fcn17/1 -> Mux1/18
  Mux/1 -> Fcn10/1, Fcn9/1, Fcn7/1, Fcn6/1, Fcn5/1, Fcn4/1, Fcn3/1, Fcn2/1, Fcn1/1, Fcn/1, Fcn14/1, Fcn15/1, Fcn16/1, Fcn17/1, Fcn18/1, Fcn13/1, Fcn12/1, Fcn11/1, Fcn8/1
  Fcn18/1 -> Mux1/19
  In11/1 -> Mux/11

== system EMT_ML/Control Unit/Control/Power Distribution/Pedal Interpretation/Brake Control ==
  Dec_pedal : Inport
  Constant : Constant  Value=0
  Fcn1 : Fcn  Expr=Fb_max*u^2
  Switch : Switch  SaturateOnIntegerOverflow=off  InputSameDT=off
  Fb_ref : Outport
  wires:
  Dec_pedal/1 -> Switch/2, Fcn1/1
  Switch/1 -> Fb_ref/1
  Fcn1/1 -> Switch/3
  Constant/1 -> Switch/1

== system EMT_ML/Control Unit/Control/Power Distribution/Pedal Interpretation/Data ==
  Dec_pedal : Inport
  Acc_pedal : Inport  Port=2
  Pe_com : Inport  Port=3
  tag scope: Acc_pedal=global, Dec_pedal=global, Pe_com=global
  wires:
  Acc_pedal/1 -> [Acc_pedal]
  Dec_pedal/1 -> [Dec_pedal]
  Pe_com/1 -> [Pe_com]

== system EMT_ML/Control Unit/Control/Power Distribution/Pedal Interpretation/Engine Power Requirement ==
  Acc_pedal : Inport
  Constant : Constant  Value=0
  Fcn : Fcn  Expr=Pe_max*u^2
  Switch1 : Switch  SaturateOnIntegerOverflow=off  InputSameDT=off
  Pe_com : Outport
  wires:
  Constant/1 -> Switch1/3
  Fcn/1 -> Switch1/1
  Acc_pedal/1 -> Switch1/2, Fcn/1
  Switch1/1 -> Pe_com/1

== system EMT_ML/Control Unit/Control/Power Distribution/Pedal Interpretation/Subsystem7 ==
  0 : Inport
  Constant : Constant  Value=0
  MinMax : MinMax  Function=max  Inputs=2
  1 : Outport
  wires:
  MinMax/1 -> 1/1
  0/1 -> MinMax/1
  Constant/1 -> MinMax/2

== system EMT_ML/Control Unit/Control/Power Distribution/Pedal Interpretation/Subsystem8 ==
  0 : Inport
  Constant : Constant  Value=0
  MinMax : MinMax  Inputs=2
  1 : Outport
  wires:
  Constant/1 -> MinMax/2
  0/1 -> MinMax/1
  MinMax/1 -> 1/1

== system EMT_ML/Control Unit/Control/Prepare Stage/clutches condition/Subsystem ==
  Constant1 : Constant
  C0 : Outport
  wires:
  Constant1/1 -> C0/1

== system EMT_ML/Control Unit/Control/Prepare Stage/clutches condition/Subsystem1 ==
  Compare To Constant1 : simulink/Logic and Bit Operations/Compare To Constant  relop=<  const=0.5  OutDataTypeStr=uint8
  Compare To Constant2 : simulink/Logic and Bit Operations/Compare To Constant  relop=<=  const=0.5  OutDataTypeStr=boolean
  Compare To Constant3 : simulink/Logic and Bit Operations/Compare To Constant  relop=<  const=Z2_shift  OutDataTypeStr=boolean
  Compare To Constant4 : simulink/Logic and Bit Operations/Compare To Constant  relop=<  const=0.5  OutDataTypeStr=uint8
  Constant : Constant  Value=ne_idl
  Data Type Conversion : DataTypeConversion  SaturateOnIntegerOverflow=off  RndMeth=Floor
  Logical Operator1 : Logic  Inputs=5  AllPortsSameDT=off  OutDataTypeStr=boolean
  Memory3 : Memory
  Memory4 : Memory
  Relational Operator : RelationalOperator  OutDataTypeStr=boolean  InputSameDT=off
  Z2 : Outport
  wires:
  Compare To Constant1/1 -> Logical Operator1/5
  Compare To Constant4/1 -> Logical Operator1/4
  [Center_Steering] -> Compare To Constant1/1
  [Generating_Knob] -> Compare To Constant4/1
  Data Type Conversion/1 -> Z2/1
  Constant/1 -> Relational Operator/2
  Compare To Constant2/1 -> Logical Operator1/3
  [Z2_rela] -> Memory3/1
  Memory3/1 -> Compare To Constant3/1
  Compare To Constant3/1 -> Logical Operator1/2
  Logical Operator1/1 -> Data Type Conversion/1
  [ne_act] -> Memory4/1
  Relational Operator/1 -> Logical Operator1/1
  Memory4/1 -> Relational Operator/1
  [Grade_Gear] -> Compare To Constant2/1

== system EMT_ML/Control Unit/Control/Prepare Stage/clutches condition/Subsystem2 ==
  Constant1 : Constant  Value=0
  C1 : Outport
  wires:
  Constant1/1 -> C1/1

== system EMT_ML/Control Unit/Control/Prepare Stage/clutches condition/Subsystem3 ==
  Compare To Constant1 : simulink/Logic and Bit Operations/Compare To Constant  relop=<  const=0.5  OutDataTypeStr=uint8
  Compare To Constant2 : simulink/Logic and Bit Operations/Compare To Constant  relop=>  const=0.5  OutDataTypeStr=boolean
  Compare To Constant3 : simulink/Logic and Bit Operations/Compare To Constant  relop=<  const=Z1_shift  OutDataTypeStr=boolean
  Compare To Constant4 : simulink/Logic and Bit Operations/Compare To Constant  relop=<  const=0.5  OutDataTypeStr=uint8
  Constant : Constant  Value=ne_idl
  Data Type Conversion : DataTypeConversion  SaturateOnIntegerOverflow=off  RndMeth=Floor
  Logical Operator1 : Logic  Inputs=5  AllPortsSameDT=off  OutDataTypeStr=boolean
  Memory2 : Memory
  Memory3 : Memory
  Relational Operator1 : RelationalOperator  OutDataTypeStr=boolean  InputSameDT=off
  Z1 : Outport
  wires:
  Compare To Constant1/1 -> Logical Operator1/5
  Compare To Constant4/1 -> Logical Operator1/4
  [Center_Steering] -> Compare To Constant1/1
  [Generating_Knob] -> Compare To Constant4/1
  Relational Operator1/1 -> Logical Operator1/1
  Constant/1 -> Relational Operator1/2
  [ne_act] -> Memory2/1
  Memory2/1 -> Relational Operator1/1
  Data Type Conversion/1 -> Z1/1
  [Grade_Gear] -> Compare To Constant2/1
  Compare To Constant2/1 -> Logical Operator1/3
  Logical Operator1/1 -> Data Type Conversion/1
  Compare To Constant3/1 -> Logical Operator1/2
  Memory3/1 -> Compare To Constant3/1
  [Z1_rela] -> Memory3/1

== system EMT_ML/Control Unit/Control/Prepare Stage/engine swich/Triggered Subsystem ==
  In1 : Inport
  Trigger : TriggerPort  VariantControl=Variant
  Out1 : Outport
  wires:
  In1/1 -> Out1/1

== system EMT_ML/Control Unit/Control/Prepare Stage/engine torque/Subsystem1 ==
  ne_act : Inport
  Constant : Constant  Value=ne_idl
  Constant1 : Constant  Value=0
  Lookup Table : Lookup  InputValues=ne_map  Table=Te_max_map  SaturateOnIntegerOverflow=off
  PID Controller2 : simulink_need_slupdate/PID Controller  P=4  I=0.01  D=10
  Saturation : Saturate  UpperLimit=max(ne_map)  LowerLimit=min(ne_map)
  Saturation Dynamic : simulink/Discontinuities/Saturation Dynamic  OutMin=[]  OutMax=[]  OutDataTypeStr=Inherit: Same as second input  OutDataType=sfix(16)  OutScaling=2^-10  DoSatur=off
  StartupFeedbackDelay : TransportDelay  DelayTime=startup_feedback_delay_s
  Sum1 : Sum  Inputs=-+
  Te_com : Outport
  wires:
  PID Controller2/1 -> Saturation Dynamic/2
  Saturation Dynamic/1 -> Te_com/1
  Constant1/1 -> Saturation Dynamic/3
  Lookup Table/1 -> Saturation Dynamic/1
  StartupFeedbackDelay/1 -> Saturation/1, Sum1/1
  ne_act/1 -> StartupFeedbackDelay/1
  Sum1/1 -> PID Controller2/1
  Saturation/1 -> Lookup Table/1
  Constant/1 -> Sum1/2
